simulink model "Horizontal1804"  (R2026b)
settings: Solver=FixedStepDiscrete  StopTime=inf  FixedStep=Official.Step
PostLoadFcn:
  | run(fullfile(fileparts(get_param('StampFly_IMU400','FileName')),'config','startup.m'));
InitFcn:
  | init_imu_flight;
undefined symbols (not defined in the file): Official
libraries: slpidlib x7, simulink x4, mspfiltlib x1
(part 2 of 5)

== system Horizontal1804/JoystickCommand ==
  BasicJoystick : MATLABSystem  Description=公式 Atom JoyStick の指令を ESP-NOW で受信します。Stick6 は [Roll, Pitch, Yaw, Thrust, 制御モード, 高度モード]。アーム、通信状態、姿勢リセット、新パケット、エラーも出力します。Flip 用ボタンは無視します。Channel は自分専用の 1～13 にし、機体のログ送信・受信機と揃えます。  Priority=5  System=basic.Joystick400  SampleTime=.0025  Channel=uint8( 3 )  SimulateUsing=Code generation
      mask Type: basic.Joystick400
  JoystickCommandBus : BusCreator  Description=JoystickCommandBus：異なる単位・型を持つ関連信号を名前付きバスにまとめます。入力線の信号名が項目名です。  Inputs=4  OutDataTypeStr=Bus: BasicLogPilotBus  NonVirtualBus=on
  RadioDiagnosticsBus : BusCreator  Description=RadioDiagnosticsBus：異なる単位・型を持つ関連信号を名前付きバスにまとめます。入力線の信号名が項目名です。  Inputs=2
  RadioDiagnosticsFields : BusSelector  Description=RadioDiagnosticsFields：バスから LinkAge,PacketError を選びます。元のベクトルの成分順序は変更しません。  OutputSignals=LinkAge,PacketError
  RawRadioAgeUnused : Terminator
      settings: Description=RawRadioAgeUnused：使用しない観測出力をここで終端します。接続された制御信号を変更しません。
  JoystickCommand : Outport
  tag scope: JoystickPacketError=global, JoystickPilot=global
  wires:
  RadioDiagnosticsBus/1 -> RadioDiagnosticsFields/1  "RadioDiagnostics"
  BasicJoystick/6 -> RadioDiagnosticsBus/2  "PacketError"
  BasicJoystick/1 -> JoystickCommandBus/1  "Sticks"
  BasicJoystick/5 -> JoystickCommandBus/3  "NewPacket"
  BasicJoystick/2 -> JoystickCommandBus/2  "ArmButton"
  BasicJoystick/3 -> RadioDiagnosticsBus/1  "LinkAge"
  JoystickCommandBus/1 -> JoystickCommand/1, [JoystickPilot]  "JoystickCommand"
  BasicJoystick/4 -> JoystickCommandBus/4  "AHRSRequest"
  RadioDiagnosticsFields/1 -> RawRadioAgeUnused/1  "<LinkAge>"
  RadioDiagnosticsFields/2 -> [JoystickPacketError]  "<PacketError>"

== system Horizontal1804/JoystickFeedback40 ==
  JapaneseExplanation : Subsystem  Description=公式 JoyStick の画面へ姿勢・高度・電池・制御状態を 40 Hz で返信します。通常ログとは別の公式 120 byte 形式です。
      mask help: 公式 JoyStick の画面へ姿勢・高度・電池・制御状態を 40 Hz で返信します。通常ログとは別の公式 120 byte 形式です。
      mask Display: disp(sprintf('公式 JoyStick の画面へ姿勢・高度・電池・制御状態を 40 Hz で返信します。\n通常ログとは別の公式 120 byte 形式です。'));
  OfficialHeaderGains20 : Constant  Description=OfficialHeaderGains20：固定値 single([.65;.7;.01;.125;.95;.7;.025;.125;3;.8;.01;.125;5;4;.04;.125;5;4;.04;.125]) を出力します。意味と単位は親の機能説明と信号名を参照します。  Value=single([.65;.7;.01;.125;.95;.7;.025;.125;3;.8;.01;.125;5;4;.04;.125;5;4;.04;.125])
  OfficialJoyTelemetry40 : MATLABSystem  Description=公式の 27 float 値とゲイン表、高度モード、飛行モード、前方距離を 40 Hz で JoyStick へ返信します。公式 120 byte 形式を保ちます。Sent は送信要求の結果です。  Priority=240  System=official.RadioTelemetryWrite40  SimulateUsing=Code generation
      mask Type: official.RadioTelemetryWrite40
  OfficialTelemetryValues : MATLAB Function  Description=JoyStick へ返す公式 120 byte テレメトリの 27 個の float 値を作ります。時刻・姿勢・目標・電池・加速度・速度・高度などを公式の単位と順序へ変換します。送信は後段の専用 I/O ブロックが行います。  TreatAsAtomicUnit=on
  Sent : Outport
  wires:
  [MotorDuty] -> OfficialTelemetryValues/8(arg_duty)
  [ControlDiagnostics] -> OfficialTelemetryValues/5(arg_cd)
  [FilteredAngularRate] -> OfficialTelemetryValues/4(arg_r)
  [AttitudeAngles] -> OfficialTelemetryValues/3(arg_a)
  [SamplePeriod] -> OfficialTelemetryValues/2(arg_dt)
  [TimeSeconds] -> OfficialTelemetryValues/1(arg_t)
  [BatteryVoltage] -> OfficialTelemetryValues/7(arg_voltage)
  [RawAcceleration] -> OfficialTelemetryValues/6(arg_accel)
  [EstimatedAltitude] -> OfficialTelemetryValues/9(arg_z)
  [SensorDiagnostics] -> OfficialTelemetryValues/10(arg_sd)
  [VerticalVelocity] -> OfficialTelemetryValues/11(arg_v)
  OfficialTelemetryValues/1(arg_values) -> OfficialJoyTelemetry40/1
  OfficialHeaderGains20/1 -> OfficialJoyTelemetry40/2
  [UnusedFrontRangeMm] -> OfficialJoyTelemetry40/5
  [AltitudeEnabled] -> OfficialJoyTelemetry40/3
  [FlightMode] -> OfficialJoyTelemetry40/4
  OfficialJoyTelemetry40/1 -> Sent/1

== system Horizontal1804/LEDAndBuzzer ==
  ControlMode : Selector  Description=ControlMode：必要なベクトル成分を選びます。選択位置は設定画面の Indices で確認します。  InputPortWidth=6  IndexOptions=Index vector (dialog)  Indices=5  OutputSizes=1
  LowVoltageCount : Selector  Description=LowVoltageCount：必要なベクトル成分を選びます。選択位置は設定画面の Indices で確認します。  InputPortWidth=3  IndexOptions=Index vector (dialog)  Indices=3  OutputSizes=1
  StatusIndicators : MATLAB Function  Description=飛行モード・電池・通信状態を LED 色とブザーへ変換します。待ち時間は 400 Hz のカウンターで管理し、機体ボタンの押下・解放を確認して再起動要求を出します。実際の LED・音・再起動は後段の I/O が行います。  TreatAsAtomicUnit=on
  StatusWrite : MATLABSystem  Description=RGB 色 2 個、ブザー周波数 [Hz]、再起動要求を機体の出力キューへ渡します。LED・音の更新は別タスクで実行します。再起動要求は機体の再起動に直結するので、状態判定ブロックからの信号を接続します。  System=official.StatusWrite400  SimulateUsing=Code generation
      mask Type: official.StatusWrite400
  UserButton : MATLABSystem  Description=StampS3 の GPIO0 ボタンを読み、押下中は uint8(1) を出力します。操縦用 JoyStick のボタンとは別です。押下時間と解放の判定は StatusIndicators で行います。  System=official.UserButton400  SimulateUsing=Code generation
      mask Type: official.UserButton400
  wires:
  [AttitudeResetRequest] -> StatusIndicators/6(arg_ahrsFlag)
  LowVoltageCount/1 -> StatusIndicators/4(arg_lowVoltage)
  [SensorFlags] -> LowVoltageCount/1
  [JoystickSticks] -> ControlMode/1
  [JoystickPacketError] -> StatusIndicators/5(arg_rcError)
  [AltitudeEnabled] -> StatusIndicators/3(arg_altFlag)
  [PreviousMode] -> StatusIndicators/1(arg_mode)
  ControlMode/1 -> StatusIndicators/2(arg_controlMode)
  UserButton/1 -> StatusIndicators/7(arg_button)
  StatusIndicators/1(arg_color1) -> StatusWrite/1
  StatusIndicators/2(arg_color2) -> StatusWrite/2
  StatusIndicators/3(arg_tone) -> StatusWrite/3
  StatusIndicators/4(arg_restart) -> StatusWrite/4

== system Horizontal1804/MagnetometerSensor ==
  DeviceRead : MATLABSystem  Description=BMM150 の補償済み磁場 XYZ [μT]、有効性・Fresh・エラー、診断を出力します。新規測定は約 30 Hz、モデルは 400 Hz で最新値を受け取ります。ToF・電池と I2C 排他を共有します。磁気は表示・記録用です。  System=stampfly.BMM150  I2CAddress=uint8( 16 )  SampleTime=.0025  SimulateUsing=Code generation
      mask Type: stampfly.BMM150
  JapaneseExplanation : Subsystem  Description=BMM150 の磁場 XYZ [μT] と有効性・Fresh・診断を取得します。センサー座標を保ってログへ渡し、姿勢推定・制御には使いません。
      mask help: BMM150 の磁場 XYZ [μT] と有効性・Fresh・診断を取得します。センサー座標を保ってログへ渡し、姿勢推定・制御には使いません。
      mask Display: disp(sprintf('BMM150 の磁場 XYZ [μT] と有効性・Fresh・診断を取得します。\nセンサー座標を保ってログへ渡し、姿勢推定・制御には使いません。'));
  SensorDataBus : BusCreator  Description=SensorDataBus：異なる単位・型を持つ関連信号を名前付きバスにまとめます。入力線の信号名が項目名です。  Inputs=3  OutDataTypeStr=Bus: LogMagBus  NonVirtualBus=on
  MagneticField : Outport
  wires:
  SensorDataBus/1 -> MagneticField/1  "SensorData"
  DeviceRead/1 -> SensorDataBus/1  "Field"
  DeviceRead/2 -> SensorDataBus/2  "Flags"
  DeviceRead/3 -> SensorDataBus/3  "Info"

== system Horizontal1804/ModelExplanation ==

== system Horizontal1804/MotorWrite ==
  MotorCommand : Inport
  JapaneseExplanation : Subsystem  Description=8 bit の Counts を実機モーターへ適用します。順序 [FR, FL, RR, RL]、GPIO [42, 5, 41, 10]、150 kHz 指定です。実適用 Counts と PWM 診断を Goto で公開します。
      mask help: 8 bit の Counts を実機モーターへ適用します。順序 [FR, FL, RR, RL]、GPIO [42, 5, 41, 10]、150 kHz 指定です。実適用 Counts と PWM 診断を Goto で公開します。
      mask Display: disp(sprintf('8 bit の Counts を実機モーターへ適用します。\n順序 [FR, FL, RR, RL]、GPIO [42, 5, 41, 10]、150 kHz 指定です。\n実適用 Counts と PWM 診断を Goto で公開します。'));
  MotorCommandFields : BusSelector  Description=MotorCommandFields：バスから Duty,Counts を選びます。元のベクトルの成分順序は変更しません。  OutputSignals=Duty,Counts
  MotorOutputEnabled : Constant  Description=MotorOutputEnabled：固定値 true を出力します。意味と単位は親の機能説明と信号名を参照します。  Value=true  SampleTime=Official.Step
  PWM150kHz8bit : MATLABSystem  Description=入力 Counts4 は [FR, FL, RR, RL] の 8 bit PWM カウントです。Enable と AllowMotorOutput が有効なとき実機へ適用し、実適用値と状態を返します。機体用は 150 kHz 指定です。これは回転数の測定値ではありません。  Priority=100  System=official.MotorPWM400  SampleTime=Official.Step  AllowMotorOutput=true  SimulateUsing=Code generation
      mask Type: official.MotorPWM400
  AppliedCounts : Outport
  PWMStatus : Outport  Port=2
  tag scope: AppliedPWMCounts=global, MotorDuty=global, PWMStatus=global
  wires:
  PWM150kHz8bit/2 -> [PWMStatus], PWMStatus/1
  MotorCommandFields/1 -> [MotorDuty]  "<Duty>"
  MotorCommand/1 -> MotorCommandFields/1
  MotorCommandFields/2 -> PWM150kHz8bit/1  "<Counts>"
  MotorOutputEnabled/1 -> PWM150kHz8bit/2
  PWM150kHz8bit/1 -> AppliedCounts/1, [AppliedPWMCounts]

== system Horizontal1804/OpticalFlowDistance50 ==
  OpticalFlow : Inport
  Attitude : Inport  Port=2
  BottomRange : Inport  Port=3
  RawIMU : Inport  Port=4
  AttitudeFields : BusSelector  Description=AttitudeFields：バスから Angles を選びます。元のベクトルの成分順序は変更しません。  OutputSignals=Angles
  DistanceData : BusCreator  Description=DistanceData：異なる単位・型を持つ関連信号を名前付きバスにまとめます。入力線の信号名が項目名です。  Inputs=3  OutDataTypeStr=Bus: LogDistanceBus  NonVirtualBus=on
  FlowFields : BusSelector  Description=FlowFields：バスから Totals,Raw を選びます。元のベクトルの成分順序は変更しません。  OutputSignals=Totals,Raw
  GroundMotionDistance : MATLABSystem  Description=400 Hz の累積カウント差を 50 Hz で集計し、姿勢・ToF・角速度を使って平らな床上の [東, 北] 移動距離 [m] に換算します。不適切な区間は位置を保持します。385 count/rad は校正前の初期値です。出力は表示・記録専用です。  System=imu.FlowDistance50  SampleTime=0.02  XCountsPerRad=385  YCountsPerRad=385  MinQuality=25  MaxHeightM=2  MaxHorizontalSpeedMps=1.5  MaxVerticalSpeedMps=2  MinDownProjection=0.5  SimulateUsing=Code generation
      mask Type: imu.FlowDistance50
  IMUFields : BusSelector  Description=IMUFields：バスから AngularRate を選びます。元のベクトルの成分順序は変更しません。  OutputSignals=AngularRate
  JapaneseExplanation : Subsystem  Description=生の累積光学フロー、姿勢、角速度、下向き ToF から平面上の東・北移動距離を 50 Hz で作ります。回転補償と品質判定を行い、無効な区間は位置を保持します。385 count/rad は初期値です。
      mask help: 生の累積光学フロー、姿勢、角速度、下向き ToF から平面上の東・北移動距離を 50 Hz で作ります。回転補償と品質判定を行い、無効な区間は位置を保持します。385 count/rad は初期値です。
      mask Display: disp(sprintf('生の累積光学フロー、姿勢、角速度、下向き ToF から平面上の東・北移動距離を 50 Hz で作ります\n。\n回転補償と品質判定を行い、無効な区間は位置を保持します。\n385 count/rad は初期値です。'));
  MillimetersToMeters : Gain  Description=MillimetersToMeters：入力に single(.001) を掛けます。座標変換・単位換算・制御係数は用途ごとに維持します。  Gain=single(.001)
  PoseAndRange4 : Mux  Description=PoseAndRange4：同じ型の値を入力端子の順でベクトルに結合します。ログ仕様・モーター順に対応する結合は順序を保ちます。  Inputs=2
  RangeFields : BusSelector  Description=RangeFields：バスから DistanceMm を選びます。元のベクトルの成分順序は変更しません。  OutputSignals=DistanceMm
  RangeToSingle : DataTypeConversion  Description=RangeToSingle：後段のバス・演算に合わせて single 型へ変換します。  OutDataTypeStr=single  SaturateOnIntegerOverflow=off  RndMeth=Floor
  FlowDistance : Outport
  wires:
  OpticalFlow/1 -> FlowFields/1  "OpticalFlow"
  RangeFields/1 -> RangeToSingle/1  "<DistanceMm>"
  BottomRange/1 -> RangeFields/1  "BottomRange"
  RawIMU/1 -> IMUFields/1  "RawIMU"
  Attitude/1 -> AttitudeFields/1  "Attitude"
  RangeToSingle/1 -> MillimetersToMeters/1
  MillimetersToMeters/1 -> PoseAndRange4/2  "ToFRangeM"
  AttitudeFields/1 -> PoseAndRange4/1  "<Angles>"
  FlowFields/1 -> GroundMotionDistance/1  "<Totals>"
  FlowFields/2 -> GroundMotionDistance/2  "<Raw>"
  IMUFields/1 -> GroundMotionDistance/3  "<AngularRate>"
  PoseAndRange4/1 -> GroundMotionDistance/4  "PoseAndRange"
  GroundMotionDistance/1 -> DistanceData/1  "PositionEN"
  GroundMotionDistance/2 -> DistanceData/2  "Used"
  GroundMotionDistance/3 -> DistanceData/3  "DeltaEN"
  DistanceData/1 -> FlowDistance/1  "FlowDistance"

== system Horizontal1804/OpticalFlowSensor ==
  DeviceRead : MATLABSystem  Description=SPI の Motion Burst から 2 軸の差分カウント、品質 Raw8、診断 Info4、巡回する累積 Totals2 を 400 Hz で取得します。カウントは距離・速度そのものではありません。距離換算は後段の FlowDistance50 で行います。  System=stampfly.PMW3901MB  SampleTime=.0025  SimulateUsing=Code generation
      mask Type: stampfly.PMW3901MB
  JapaneseExplanation : Subsystem  Description=PMW3901 の生 2 軸差分・品質・診断・累積カウントを取得します。表示・記録専用で、水平位置制御へは戻しません。
      mask help: PMW3901 の生 2 軸差分・品質・診断・累積カウントを取得します。表示・記録専用で、水平位置制御へは戻しません。
      mask Display: disp(sprintf('PMW3901 の生 2 軸差分・品質・診断・累積カウントを取得します。\n表示・記録専用で、水平位置制御へは戻しません。'));
  SensorDataBus : BusCreator  Description=SensorDataBus：異なる単位・型を持つ関連信号を名前付きバスにまとめます。入力線の信号名が項目名です。  Inputs=4  OutDataTypeStr=Bus: LogFlowBus  NonVirtualBus=on
  OpticalFlow : Outport
  wires:
  DeviceRead/1 -> SensorDataBus/1  "Delta"
  DeviceRead/2 -> SensorDataBus/2  "Raw"
  DeviceRead/3 -> SensorDataBus/3  "Info"
  DeviceRead/4 -> SensorDataBus/4  "Totals"
  SensorDataBus/1 -> OpticalFlow/1  "SensorData"

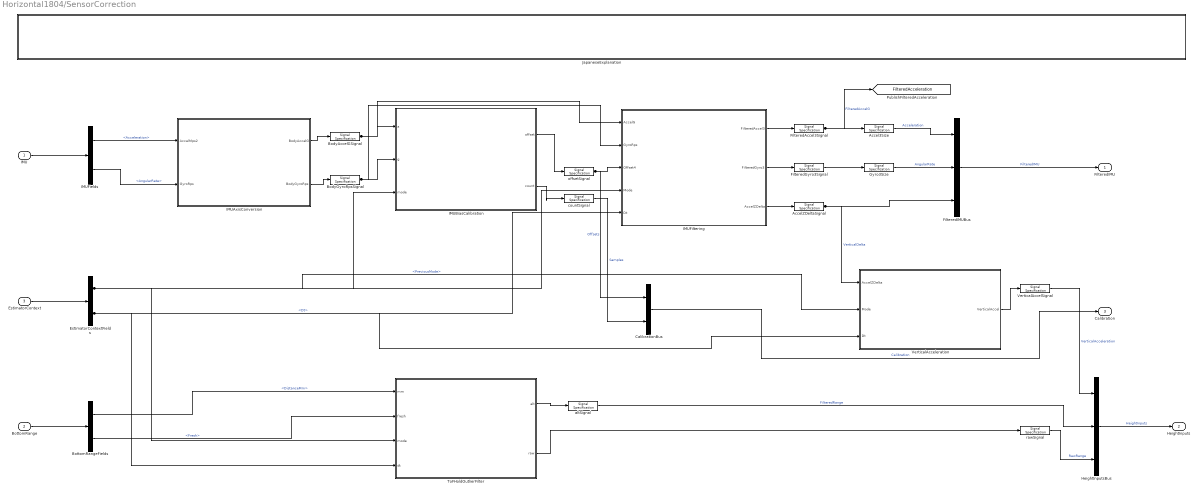
== system Horizontal1804/SensorCorrection ==
  IMU : Inport
  BottomRange : Inport  Port=2
  EstimatorContext : Inport  Port=3
  Accel3Size : SignalSpecification  OutDataTypeStr=single  Dimensions=3
  AccelZDeltaSignal : SignalSpecification  OutDataTypeStr=single  Dimensions=1
  BodyAccelGSignal : SignalSpecification  OutDataTypeStr=single  Dimensions=3
  BodyGyroRpsSignal : SignalSpecification  OutDataTypeStr=single  Dimensions=3
  BottomRangeFields : BusSelector  Description=BottomRangeFields：バスから DistanceMm,Fresh を選びます。元のベクトルの成分順序は変更しません。  OutputSignals=DistanceMm,Fresh
  CalibrationBus : BusCreator  Description=CalibrationBus：異なる単位・型を持つ関連信号を名前付きバスにまとめます。入力線の信号名が項目名です。  Inputs=2
  EstimatorContextFields : BusSelector  Description=EstimatorContextFields：バスから PreviousMode,Dt を選びます。元のベクトルの成分順序は変更しません。  OutputSignals=PreviousMode,Dt
  FilteredAccel3Signal : SignalSpecification  OutDataTypeStr=single  Dimensions=3
  FilteredGyro3Signal : SignalSpecification  OutDataTypeStr=single  Dimensions=3
  FilteredIMUBus : BusCreator  Description=FilteredIMUBus：異なる単位・型を持つ関連信号を名前付きバスにまとめます。入力線の信号名が項目名です。  Inputs=3
  Gyro3Size : SignalSpecification  OutDataTypeStr=single  Dimensions=3
  HeightInputsBus : BusCreator  Description=HeightInputsBus：異なる単位・型を持つ関連信号を名前付きバスにまとめます。入力線の信号名が項目名です。  Inputs=3
  IMUAxisConversion : Subsystem  Description=センサー XYZ を機体 [Y, X, -Z] へ変換します。加速度を m/s² から g 基準へ換算し、角速度は rad/s を保ちます。この座標変換はセンサーの取り付けと既存制御の定義に必要です。
      mask help: センサー XYZ を機体 [Y, X, -Z] へ変換します。加速度を m/s² から g 基準へ換算し、角速度は rad/s を保ちます。この座標変換はセンサーの取り付けと既存制御の定義に必要です。
      mask Display: disp('IMUAxisConversion');port_label('input',1,'AccelMps2');port_label('input',2,'GyroRps');port_label('output',1,'BodyAccelG');port_label('output',2,'BodyGyroRps');
  IMUBiasCalibration : MATLAB Function  Description=起動時に静止した機体のジャイロ XYZ と加速度 Z を 800 周期平均します。出力 Offset は [GyroX; GyroY; GyroZ; AccelZ]、Count は取得数です。400 Hz で公称 2 秒の校正中は機体を動かさないでください。  TreatAsAtomicUnit=on
  IMUFields : BusSelector  Description=IMUFields：バスから Acceleration,AngularRate を選びます。元のベクトルの成分順序は変更しません。  OutputSignals=Acceleration,AngularRate
  IMUFiltering : Subsystem  Description=加速度と校正後角速度の XYZ ベクトルを時定数 3 ms で低域フィルターに通します。Z 加速度の校正差分は 100 ms で処理します。Mode 0, 1 の保持、待機への移行時リセット、実測 dt と既存の演算順序を維持します。
      mask help: 加速度と校正後角速度の XYZ ベクトルを時定数 3 ms で低域フィルターに通します。Z 加速度の校正差分は 100 ms で処理します。Mode 0, 1 の保持、待機への移行時リセット、実測 dt と既存の演算順序を維持します。
      mask Display: disp('IMUFiltering');port_label('input',1,'AccelG');port_label('input',2,'GyroRps');port_label('input',3,'Offset4');port_label('input',4,'Mode');port_label('input',5,'Dt');port_label('output',1,'FilteredAccel3');port_label('output',2,'FilteredGyro3');port_label('output',3,'AccelZDelta');
  JapaneseExplanation : Subsystem  Description=センサー座標から機体 XYZ へ変換し、800 周期の静止校正とフィルターを行います。加速度 XYZ・角速度 XYZ の順を維持し、ToF の保持・外れ値処理と鉛直加速度もまとめます。推定用の前処理は Mode 0, 1 で保持します。
      mask help: センサー座標から機体 XYZ へ変換し、800 周期の静止校正とフィルターを行います。加速度 XYZ・角速度 XYZ の順を維持し、ToF の保持・外れ値処理と鉛直加速度もまとめます。推定用の前処理は Mode 0, 1 で保持します。
      mask Display: disp(sprintf('センサー座標から機体 XYZ へ変換し、800 周期の静止校正とフィルターを行います。\n加速度 XYZ・角速度 XYZ の順を維持し、ToF の保持・外れ値処理と鉛直加速度もまとめます。\n推定用の前処理は Mode 0, 1 で保持します。'));
  ToFHoldOutlierFilter : MATLAB Function  Description=新しい下向き距離 [mm] を保持・外れ値処理して高さ [m] へ変換します。20 mm 以下は前回の有効距離を使い、500 mm 超の飛びは最大 2 回まで履歴から補外します。Mode 0, 1 では推定用の出力を保持します。  TreatAsAtomicUnit=on
  VerticalAccelSignal : SignalSpecification  OutDataTypeStr=single  Dimensions=1
  VerticalAcceleration : Subsystem  Description=校正後の Z 加速度差分の符号を反転し、上向きの鉛直加速度を作ります。100 ms の平滑化とモードによる保持・リセットを行います。高度 Kalman は従来の g 基準の数値を受けます。
      mask help: 校正後の Z 加速度差分の符号を反転し、上向きの鉛直加速度を作ります。100 ms の平滑化とモードによる保持・リセットを行います。高度 Kalman は従来の g 基準の数値を受けます。
      mask Display: disp('VerticalAcceleration');port_label('input',1,'AccelZDelta');port_label('input',2,'Mode');port_label('input',3,'Dt');port_label('output',1,'VerticalAccel');
  altSignal : SignalSpecification  OutDataTypeStr=single  Dimensions=1
  countSignal : SignalSpecification  OutDataTypeStr=uint16  Dimensions=1
  offsetSignal : SignalSpecification  OutDataTypeStr=single  Dimensions=4
  rawSignal : SignalSpecification  OutDataTypeStr=int16  Dimensions=1
  FilteredIMU : Outport
  HeightInputs : Outport  Port=2
  Calibration : Outport  Port=3
  tag scope: FilteredAcceleration=global
  wires:
  EstimatorContext/1 -> EstimatorContextFields/1
  BottomRangeFields/2 -> ToFHoldOutlierFilter/2(fresh)  "<Fresh>"
  IMUAxisConversion/2(BodyGyroRps) -> BodyGyroRpsSignal/1
  IMU/1 -> IMUFields/1
  IMUBiasCalibration/2(count) -> countSignal/1
  IMUFields/1 -> IMUAxisConversion/1(AccelMps2)  "<Acceleration>"
  IMUFields/2 -> IMUAxisConversion/2(GyroRps)  "<AngularRate>"
  BottomRangeFields/1 -> ToFHoldOutlierFilter/1(mm)  "<DistanceMm>"
  IMUAxisConversion/1(BodyAccelG) -> BodyAccelGSignal/1
  FilteredGyro3Signal/1 -> Gyro3Size/1
  BottomRange/1 -> BottomRangeFields/1
  BodyAccelGSignal/1 -> IMUFiltering/1(AccelG), IMUBiasCalibration/1(a)
  HeightInputsBus/1 -> HeightInputs/1  "HeightInputs"
  BodyGyroRpsSignal/1 -> IMUFiltering/2(GyroRps), IMUBiasCalibration/2(g)
  EstimatorContextFields/1 -> IMUFiltering/4(Mode), VerticalAcceleration/2(Mode), ToFHoldOutlierFilter/3(mode), IMUBiasCalibration/3(mode)  "<PreviousMode>"
  EstimatorContextFields/2 -> VerticalAcceleration/3(Dt), IMUFiltering/5(Dt), ToFHoldOutlierFilter/4(dt)  "<Dt>"
  IMUBiasCalibration/1(offset) -> offsetSignal/1
  ToFHoldOutlierFilter/1(alt) -> altSignal/1
  Gyro3Size/1 -> FilteredIMUBus/2  "AngularRate"
  AccelZDeltaSignal/1 -> VerticalAcceleration/1(AccelZDelta), FilteredIMUBus/3  "VerticalDelta"
  ToFHoldOutlierFilter/2(raw) -> rawSignal/1
  countSignal/1 -> CalibrationBus/2  "Samples"
  offsetSignal/1 -> IMUFiltering/3(Offset4), CalibrationBus/1  "Offsets"
  CalibrationBus/1 -> Calibration/1  "Calibration"
  altSignal/1 -> HeightInputsBus/2  "FilteredRange"
  IMUFiltering/1(FilteredAccel3) -> FilteredAccel3Signal/1
  IMUFiltering/2(FilteredGyro3) -> FilteredGyro3Signal/1
  IMUFiltering/3(AccelZDelta) -> AccelZDeltaSignal/1
  VerticalAccelSignal/1 -> HeightInputsBus/1  "VerticalAcceleration"
  rawSignal/1 -> HeightInputsBus/3  "RawRange"
  FilteredAccel3Signal/1 -> [FilteredAcceleration], Accel3Size/1  "FilteredAccelG"
  VerticalAcceleration/1(VerticalAccel) -> VerticalAccelSignal/1
  Accel3Size/1 -> FilteredIMUBus/1  "Acceleration"
  FilteredIMUBus/1 -> FilteredIMU/1  "FilteredIMU"

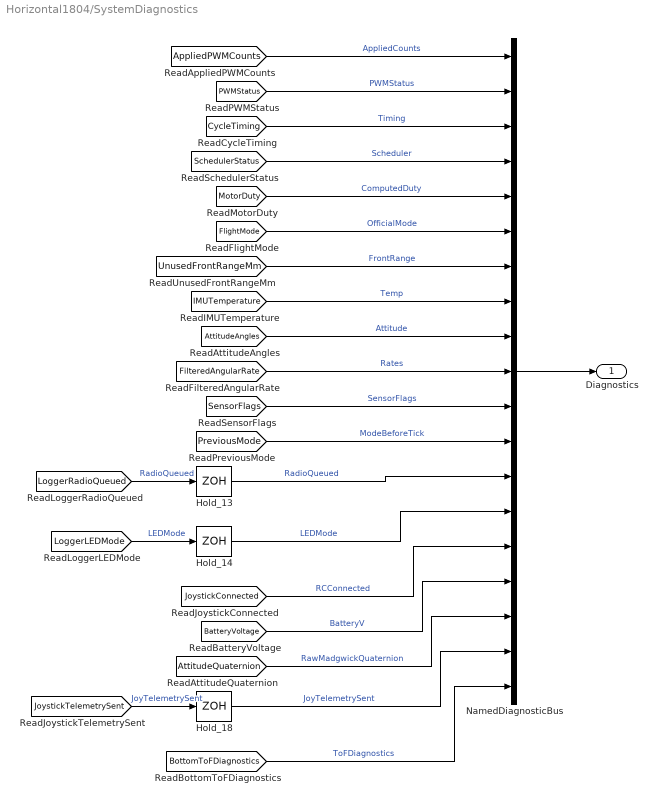
== system Horizontal1804/SystemDiagnostics ==
  Hold_13 : ZeroOrderHold  Description=Hold_13：入力の最新値を指定周期で保持します。異なる更新周期の観測値を診断へ渡します。  SampleTime=.0025
  Hold_14 : ZeroOrderHold  Description=Hold_14：入力の最新値を指定周期で保持します。異なる更新周期の観測値を診断へ渡します。  SampleTime=.0025
  Hold_18 : ZeroOrderHold  Description=Hold_18：入力の最新値を指定周期で保持します。異なる更新周期の観測値を診断へ渡します。  SampleTime=.0025
  NamedDiagnosticBus : BusCreator  Description=NamedDiagnosticBus：異なる単位・型を持つ関連信号を名前付きバスにまとめます。入力線の信号名が項目名です。  Inputs=19  OutDataTypeStr=Bus: OfficialDiagnosticBus  NonVirtualBus=on
  Diagnostics : Outport
  wires:
  [SchedulerStatus] -> NamedDiagnosticBus/4  "Scheduler"
  [AppliedPWMCounts] -> NamedDiagnosticBus/1  "AppliedCounts"
  [LoggerRadioQueued] -> Hold_13/1  "RadioQueued"
  [LoggerLEDMode] -> Hold_14/1  "LEDMode"
  [PWMStatus] -> NamedDiagnosticBus/2  "PWMStatus"
  [JoystickTelemetrySent] -> Hold_18/1  "JoyTelemetrySent"
  [MotorDuty] -> NamedDiagnosticBus/5  "ComputedDuty"
  [CycleTiming] -> NamedDiagnosticBus/3  "Timing"
  [FlightMode] -> NamedDiagnosticBus/6  "OfficialMode"
  [UnusedFrontRangeMm] -> NamedDiagnosticBus/7  "FrontRange"
  [IMUTemperature] -> NamedDiagnosticBus/8  "Temp"
  [AttitudeAngles] -> NamedDiagnosticBus/9  "Attitude"
  [FilteredAngularRate] -> NamedDiagnosticBus/10  "Rates"
  [SensorFlags] -> NamedDiagnosticBus/11  "SensorFlags"
  [PreviousMode] -> NamedDiagnosticBus/12  "ModeBeforeTick"
  Hold_13/1 -> NamedDiagnosticBus/13  "RadioQueued"
  Hold_14/1 -> NamedDiagnosticBus/14  "LEDMode"
  [JoystickConnected] -> NamedDiagnosticBus/15  "RCConnected"
  [BatteryVoltage] -> NamedDiagnosticBus/16  "BatteryV"
  [AttitudeQuaternion] -> NamedDiagnosticBus/17  "RawMadgwickQuaternion"
  Hold_18/1 -> NamedDiagnosticBus/18  "JoyTelemetrySent"
  [BottomToFDiagnostics] -> NamedDiagnosticBus/19  "ToFDiagnostics"
  NamedDiagnosticBus/1 -> Diagnostics/1

== system Horizontal1804/TickStart ==
  CycleClock : MATLABSystem  Description=2500 μs の GPTimer で制御タスクを起動し、開始時刻 [μs]、実測 dt [s]、タイマー診断を返します。モデルの Fixed-step も 0.0025 秒に揃えます。生成された step の計測設定はモデル名 StampFly_IMU400 に対応しています。  Priority=1  System=official.TickStart400  SampleTime=Official.Step  SimulateUsing=Code generation
      mask Type: official.TickStart400
  UsToSeconds : Gain  Description=UsToSeconds：入力に single(1e-6) を掛けます。座標変換・単位換算・制御係数は用途ごとに維持します。  Gain=single(1e-6)  OutDataTypeStr=single
  Dt : Outport
  tag scope: CycleStartUs=global, SamplePeriod=global, SchedulerStatus=global, TimeSeconds=global
  wires:
  CycleClock/1 -> [CycleStartUs], UsToSeconds/1  "StartUs"
  CycleClock/2 -> Dt/1, [SamplePeriod]
  CycleClock/3 -> [SchedulerStatus]
  UsToSeconds/1 -> [TimeSeconds]

== system Horizontal1804/AttitudeAltitudeEstimation/IMUAttitude ==
  AngularRate : Inport
  AccelerationG : Inport  Port=2
  PreviousMode : Inport  Port=3
  AttitudeReset : Inport  Port=4
  FilterInputs : MATLAB Function  Description=IMU Filter の入力を準備します。機体座標 XYZ の角速度 [rad/s] と加速度 [g] を、推定器の座標と SI 単位へ変換します。校正中のリセット要求は、推定を再開するまで保持します。  TreatAsAtomicUnit=on
  FlightOutputs : MATLAB Function  Description=IMU Filter の姿勢とバイアス補正済み角速度を、従来の飛行制御の座標・順序へ戻します。出力は角度 [Roll, Pitch, Yaw] [rad]、クォータニオン [w, x, y, z]、機体 XYZ 角速度 [rad/s] です。  TreatAsAtomicUnit=on
  FusionState : Subsystem  Description=Mode 0, 1 では IMU Filter の予測・補正を実行せず状態を保持する Enabled subsystem です。停止中のリセットは FilterInputs が記憶し、再開時に内部へ渡します。  TreatAsAtomicUnit=on
      mask help: Mode 0, 1 では IMU Filter の予測・補正を実行せず状態を保持する Enabled subsystem です。停止中のリセットは FilterInputs が記憶し、再開時に内部へ渡します。
      mask Display: disp('FusionState');port_label('input',1,'Accel');port_label('input',2,'Gyro');port_label('input',3,'Reset');port_label('output',1,'Orientation');port_label('output',2,'AngularVelocity');
  Angles : Outport
  Quaternion : Outport  Port=2
  CorrectedAngularRate : Outport  Port=3
  wires:
  AngularRate/1 -> FlightOutputs/5(rawRates), FilterInputs/1(rates)
  AccelerationG/1 -> FilterInputs/2(accelG)
  FilterInputs/4(filterReset) -> FusionState/3(Reset)  "PendingReset"
  AttitudeReset/1 -> FilterInputs/4(reset), FlightOutputs/4(reset)
  FilterInputs/3(run) -> FusionState/Enable, FlightOutputs/3(run)
  FilterInputs/2(gyroRps) -> FusionState/2(Gyro)  "GyroRps"
  PreviousMode/1 -> FilterInputs/3(mode)
  FilterInputs/1(accelMps2) -> FusionState/1(Accel)  "AccelMps2"
  FusionState/1(Orientation) -> FlightOutputs/1(orientation)
  FusionState/2(AngularVelocity) -> FlightOutputs/2(angularVelocity)
  FlightOutputs/1(angles) -> Angles/1  "Angles"
  FlightOutputs/2(q) -> Quaternion/1  "Quaternion"
  FlightOutputs/3(rates) -> CorrectedAngularRate/1  "AngularRate"

== system Horizontal1804/AttitudeAltitudeEstimation/JapaneseExplanation ==

== system Horizontal1804/BottomRangeSensor/JapaneseExplanation ==

== system Horizontal1804/CommandPreparation/JapaneseExplanation ==

== system Horizontal1804/DataLogging50/JapaneseExplanation ==

== system Horizontal1804/EstimatorContext/JapaneseExplanation ==

== system Horizontal1804/FlightControl/JapaneseExplanation ==

== system Horizontal1804/FlightControl/PreviousCycle ==
  ControlState : Inport
  SupervisorReset : Inport  Port=2
  AHRSResetMemory : UnitDelay  Description=AHRSResetMemory：前周期の値を保持して出力します。更新順序と状態保持に必要な 1 周期遅延です。初期値 false、周期 Official.Step 秒。  InitialCondition=false  SampleTime=Official.Step
  AltFlagMemory : UnitDelay  Description=AltFlagMemory：前周期の値を保持して出力します。更新順序と状態保持に必要な 1 周期遅延です。初期値 uint8(0)、周期 Official.Step 秒。  InitialCondition=uint8(0)  SampleTime=Official.Step
  AltFlagUInt8 : DataTypeConversion  Description=AltFlagUInt8：後段のバス・演算に合わせて uint8 型へ変換します。  OutDataTypeStr=uint8  SaturateOnIntegerOverflow=off  RndMeth=Floor
  ControlStateFields : BusSelector  Description=ControlStateFields：バスから AltitudeEnabled,Mode を選びます。元のベクトルの成分順序は変更しません。  OutputSignals=AltitudeEnabled,Mode
  EstimatorFeedbackBus : BusCreator  Description=EstimatorFeedbackBus：異なる単位・型を持つ関連信号を名前付きバスにまとめます。入力線の信号名が項目名です。  Inputs=4
  ModeMemory : UnitDelay  Description=ModeMemory：前周期の値を保持して出力します。更新順序と状態保持に必要な 1 周期遅延です。初期値 uint8(0)、周期 Official.Step 秒。  InitialCondition=uint8(0)  SampleTime=Official.Step
  ParkingResetMemory : UnitDelay  Description=ParkingResetMemory：前周期の値を保持して出力します。更新順序と状態保持に必要な 1 周期遅延です。初期値 false、周期 Official.Step 秒。  InitialCondition=false  SampleTime=Official.Step
  SupervisorResetFields : BusSelector  Description=SupervisorResetFields：バスから AttitudeReset,ParkingReset を選びます。元のベクトルの成分順序は変更しません。  OutputSignals=AttitudeReset,ParkingReset
  EstimatorFeedback : Outport
  PreviousMode : Outport  Port=2
  AltitudeEnabled : Outport  Port=3
  wires:
  ControlStateFields/1 -> AltFlagUInt8/1  "<AltitudeEnabled>"
  SupervisorResetFields/1 -> AHRSResetMemory/1  "<AttitudeReset>"
  AltFlagMemory/1 -> EstimatorFeedbackBus/2  "AltitudeEnabled"
  ModeMemory/1 -> EstimatorFeedbackBus/1, PreviousMode/1  "PreviousMode"
  SupervisorReset/1 -> SupervisorResetFields/1
  ControlState/1 -> ControlStateFields/1
  ControlStateFields/2 -> ModeMemory/1  "<Mode>"
  SupervisorResetFields/2 -> ParkingResetMemory/1  "<ParkingReset>"
  ParkingResetMemory/1 -> EstimatorFeedbackBus/4  "ParkingReset"
  AltFlagUInt8/1 -> AltFlagMemory/1, AltitudeEnabled/1  "AltitudeEnabled"
  EstimatorFeedbackBus/1 -> EstimatorFeedback/1  "EstimatorFeedback"
  AHRSResetMemory/1 -> EstimatorFeedbackBus/3  "AttitudeReset"

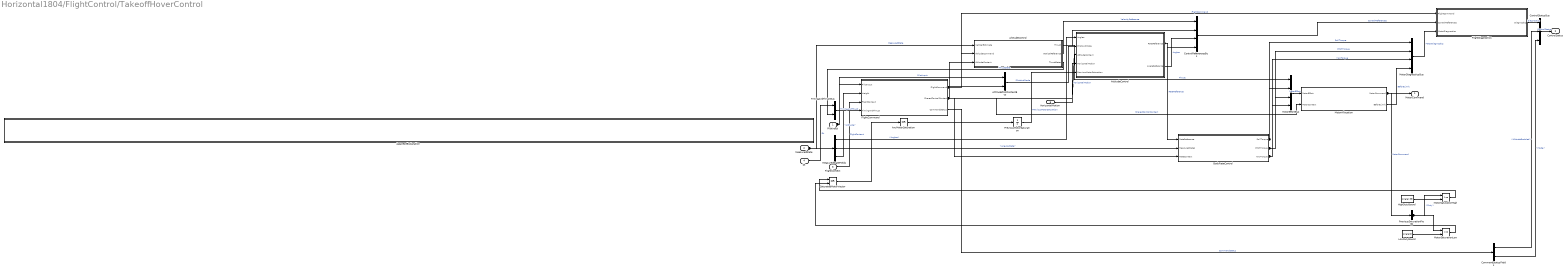
== system Horizontal1804/FlightControl/TakeoffHoverControl ==
  PilotInput : Inport
  MeasuredState : Inport  Port=2
  FlightContext : Inport  Port=3
  Dt : Inport  Port=4
  HorizontalMotion : Inport  Description=HorizontalMotion：水平推定・制御のデータと実行条件を選択・結合します。2軸の順序は局所X（基準機首）、Y（右）です。  Port=5  OutDataTypeStr=Bus: HorizontalMotionBus
  AltitudeControl : Subsystem  Description=高度誤差を高度 PID で目標鉛直速度へ変換し、鉛直速度 PID で共通推力を補正します。自動高度と着陸降下を選び、平滑化と推力制限を行います。
      mask help: 高度誤差を高度 PID で目標鉛直速度へ変換し、鉛直速度 PID で共通推力を補正します。自動高度と着陸降下を選び、平滑化と推力制限を行います。
      mask Display: disp('AltitudeControl');port_label('input',1,'VerticalEstimate');port_label('input',2,'AltitudeCommand');port_label('input',3,'AltitudeContext');port_label('output',1,'Thrust');port_label('output',2,'VerticalReference');port_label('output',3,'ThrustState');
  AnyMotorSaturation : Logic  Description=AnyMotorSaturation：水平推定・制御のデータと実行条件を選択・結合します。2軸の順序は局所X（基準機首）、Y（右）です。  Operator=OR  Inputs=1  IconShape=distinctive  AllPortsSameDT=off  OutDataTypeStr=boolean
  AttitudeControl : Subsystem  Description=Stabilize の Roll/Pitch 角度誤差を角度 PID へ渡して角速度目標を作ります。Sport は直接角速度目標を使い、Yaw の指令は角度ループを通しません。
      mask help: Stabilize の Roll/Pitch 角度誤差を角度 PID へ渡して角速度目標を作ります。Sport は直接角速度目標を使い、Yaw の指令は角度ループを通しません。
      mask Display: disp('AttitudeControl');port_label('input',1,'Angles');port_label('input',2,'PilotAndMode');port_label('input',3,'AttitudeContext');port_label('input',4,'HorizontalMotion');port_label('input',5,'PreviousMotorSaturation');port_label('output',1,'RateReference');port_label('output',2,'AngleReference');
  AttitudePilotContextBus : BusCreator  Description=AttitudePilotContextBus：異なる単位・型を持つ関連信号を名前付きバスにまとめます。入力線の信号名が項目名です。  Inputs=2
  BodyRateControl : Subsystem  Description=Roll/Pitch/Yaw の目標と推定角速度との差を各 PID で処理し、モーターに加える 3 軸の補正を作ります。角速度は機体 XYZ、rad/s です。
      mask help: Roll/Pitch/Yaw の目標と推定角速度との差を各 PID で処理し、モーターに加える 3 軸の補正を作ります。角速度は機体 XYZ、rad/s です。
      mask Display: disp('BodyRateControl');port_label('input',1,'RateReference');port_label('input',2,'MeasuredRates');port_label('input',3,'RateContext');port_label('output',1,'RollTorque');port_label('output',2,'PitchTorque');port_label('output',3,'YawTorque');
  CommandStatusFields : BusSelector  Description=CommandStatusFields：バスから AltitudeEnabled,Mode を選びます。元のベクトルの成分順序は変更しません。  OutputSignals=AltitudeEnabled,Mode
  ControlReferencesBus : BusCreator  Description=ControlReferencesBus：異なる単位・型を持つ関連信号を名前付きバスにまとめます。入力線の信号名が項目名です。  Inputs=4
  ControlStatusBus : BusCreator  Description=ControlStatusBus：異なる単位・型を持つ関連信号を名前付きバスにまとめます。入力線の信号名が項目名です。  Inputs=3
  FlightCommand : Subsystem  Description=スティック、高度目標、離着陸カウンター、共通推力とモードを決めます。低推力条件に応じた制御ループの許可・リセットも生成します。
      mask help: スティック、高度目標、離着陸カウンター、共通推力とモードを決めます。低推力条件に応じた制御ループの許可・リセットも生成します。
      mask Display: disp('FlightCommand');port_label('input',1,'PilotInput');port_label('input',2,'Height');port_label('input',3,'FlightContext');port_label('input',4,'TimingAndThrust');port_label('output',1,'FlightCommand');port_label('output',2,'SharedControlContext');port_label('output',3,'CommandStatus');
  FlightDiagnostics : Subsystem  Description=高度目標、推力、角度・角速度目標、3 軸補正、配分前値をログの既存 17 要素順序へまとめます。制御の判断は行いません。
      mask help: 高度目標、推力、角度・角速度目標、3 軸補正、配分前値をログの既存 17 要素順序へまとめます。制御の判断は行いません。
      mask Display: disp('FlightDiagnostics');port_label('input',1,'FlightCommand');port_label('input',2,'ControlReferences');port_label('input',3,'MotorDiagnostics');port_label('output',1,'Diagnostics');
  HighDutyBound : Constant  Description=HighDutyBound：水平推定・制御のデータと実行条件を選択・結合します。2軸の順序は局所X（基準機首）、Y（右）です。  Value=single(.95)
  JapaneseExplanation : Subsystem  Description=離着陸・高度制御・姿勢制御・角速度制御・モーター配分を機能別にまとめます。高度→速度、角度→角速度の二重ループを読みます。
      mask help: 離着陸・高度制御・姿勢制御・角速度制御・モーター配分を機能別にまとめます。高度→速度、角度→角速度の二重ループを読みます。
      mask Display: disp(sprintf('離着陸・高度制御・姿勢制御・角速度制御・モーター配分を機能別にまとめます。\n高度→速度、角度→角速度の二重ループを読みます。'));
  LowDutyBound : Constant  Description=LowDutyBound：水平推定・制御のデータと実行条件を選択・結合します。2軸の順序は局所X（基準機首）、Y（右）です。  Value=single(0)
  MeasuredStateFields : BusSelector  Description=MeasuredStateFields：バスから Angles,AngularRate,Altitude を選びます。元のベクトルの成分順序は変更しません。  OutputSignals=Angles,AngularRate,Altitude
  MotorAllocation : Subsystem  Description=共通推力と 3 軸の補正を [FR, FL, RR, RL] の 4 モーターへ配分します。3 ms 平滑化、Duty 0～0.95 の制限、floor(255*Duty) の量子化を行います。
      mask help: 共通推力と 3 軸の補正を [FR, FL, RR, RL] の 4 モーターへ配分します。3 ms 平滑化、Duty 0～0.95 の制限、floor(255*Duty) の量子化を行います。
      mask Display: disp('MotorAllocation');port_label('input',1,'MotorEffort');port_label('input',2,'MotorContext');port_label('output',1,'MotorCommand');port_label('output',2,'BeforeLimit');
  MotorDiagnosticsBus : BusCreator  Description=MotorDiagnosticsBus：異なる単位・型を持つ関連信号を名前付きバスにまとめます。入力線の信号名が項目名です。  Inputs=4
  MotorEffortBus : BusCreator  Description=MotorEffortBus：異なる単位・型を持つ関連信号を名前付きバスにまとめます。入力線の信号名が項目名です。  Inputs=4
  MotorSaturationHigh : RelationalOperator  Description=MotorSaturationHigh：水平推定・制御のデータと実行条件を選択・結合します。2軸の順序は局所X（基準機首）、Y（右）です。  OutDataTypeStr=boolean  RndMeth=Simplest  InputSameDT=off
  MotorSaturationLow : RelationalOperator  Description=MotorSaturationLow：水平推定・制御のデータと実行条件を選択・結合します。2軸の順序は局所X（基準機首）、Y（右）です。  Operator=<=  OutDataTypeStr=boolean  RndMeth=Simplest  InputSameDT=off
  PreviousMotorSaturation : UnitDelay  Description=PreviousMotorSaturation：水平推定・制御のデータと実行条件を選択・結合します。2軸の順序は局所X（基準機首）、Y（右）です。  InitialCondition=false  SampleTime=Official.Step
  PreviousSaturationFields : BusSelector  Description=PreviousSaturationFields：水平推定・制御のデータと実行条件を選択・結合します。2軸の順序は局所X（基準機首）、Y（右）です。  OutputSignals=Duty
  SaturatedMotorVector : Logic  Description=SaturatedMotorVector：水平推定・制御のデータと実行条件を選択・結合します。2軸の順序は局所X（基準機首）、Y（右）です。  Operator=OR  IconShape=distinctive  AllPortsSameDT=off  OutDataTypeStr=boolean
  TimingAndThrustBus : BusCreator  Description=TimingAndThrustBus：異なる単位・型を持つ関連信号を名前付きバスにまとめます。入力線の信号名が項目名です。  Inputs=2
  MotorCommand : Outport
  ControlStatus : Outport  Port=2
  wires:
  PilotInput/1 -> AttitudePilotContextBus/1, FlightCommand/1(PilotInput)  "PilotInput"
  MeasuredState/1 -> AltitudeControl/1(VerticalEstimate), MeasuredStateFields/1  "MeasuredState"
  AnyMotorSaturation/1 -> PreviousMotorSaturation/1
  SaturatedMotorVector/1 -> AnyMotorSaturation/1
  FlightContext/1 -> FlightCommand/3(FlightContext)  "FlightContext"
  HighDutyBound/1 -> MotorSaturationHigh/2
  MotorDiagnosticsBus/1 -> FlightDiagnostics/3(MotorDiagnostics)  "MotorDiagnostics"
  HorizontalMotion/1 -> AttitudeControl/4(HorizontalMotion)  "HorizontalMotion"
  MeasuredStateFields/3 -> FlightCommand/2(Height)  "<Altitude>"
  Dt/1 -> TimingAndThrustBus/1  "Dt"
  TimingAndThrustBus/1 -> FlightCommand/4(TimingAndThrust)  "TimingAndThrust"
  MeasuredStateFields/1 -> AttitudeControl/1(Angles)  "<Angles>"
  MeasuredStateFields/2 -> BodyRateControl/2(MeasuredRates)  "<AngularRate>"
  FlightCommand/1(FlightCommand) -> FlightDiagnostics/1(FlightCommand), AltitudeControl/2(AltitudeCommand)  "FlightCommand"
  AttitudeControl/1(RateReference) -> BodyRateControl/1(RateReference), ControlReferencesBus/4  "RateReference"
  AltitudeControl/2(VerticalReference) -> ControlReferencesBus/1  "VelocityReference"
  FlightCommand/2(SharedControlContext) -> BodyRateControl/3(RateContext), MotorAllocation/2(MotorContext), AttitudePilotContextBus/2, AltitudeControl/3(AltitudeContext), AttitudeControl/3(AttitudeContext)  "SharedControlContext"
  FlightCommand/3(CommandStatus) -> CommandStatusFields/1  "CommandStatus"
  MotorSaturationHigh/1 -> SaturatedMotorVector/1
  AttitudeControl/2(AngleReference) -> ControlReferencesBus/3  "Angles"
  AltitudeControl/1(Thrust) -> MotorEffortBus/1, ControlReferencesBus/2  "Thrust"
  MotorSaturationLow/1 -> SaturatedMotorVector/2
  AltitudeControl/3(ThrustState) -> TimingAndThrustBus/2  "ThrustState"
  CommandStatusFields/1 -> ControlStatusBus/2  "<AltitudeEnabled>"
  AttitudePilotContextBus/1 -> AttitudeControl/2(PilotAndMode)  "PilotAndMode"
  LowDutyBound/1 -> MotorSaturationLow/2
  BodyRateControl/3(YawTorque) -> MotorDiagnosticsBus/3, MotorEffortBus/4  "YawTorque"
  PreviousMotorSaturation/1 -> AttitudeControl/5(PreviousMotorSaturation)  "PreviousMotorSaturation"
  ControlReferencesBus/1 -> FlightDiagnostics/2(ControlReferences)  "ControlReferences"
  BodyRateControl/1(RollTorque) -> MotorDiagnosticsBus/1, MotorEffortBus/2  "RollTorque"
  BodyRateControl/2(PitchTorque) -> MotorDiagnosticsBus/2, MotorEffortBus/3  "PitchTorque"
  MotorEffortBus/1 -> MotorAllocation/1(MotorEffort)  "MotorEffort"
  MotorAllocation/1(MotorCommand) -> MotorCommand/1, PreviousSaturationFields/1  "MotorCommand"
  MotorAllocation/2(BeforeLimit) -> MotorDiagnosticsBus/4  "BeforeLimit"
  PreviousSaturationFields/1 -> MotorSaturationHigh/1, MotorSaturationLow/1  "<Duty>"
  FlightDiagnostics/1(Diagnostics) -> ControlStatusBus/1  "Diagnostics"
  CommandStatusFields/2 -> ControlStatusBus/3  "<Mode>"
  ControlStatusBus/1 -> ControlStatus/1  "ControlStatus"

== system Horizontal1804/IMUSensor/JapaneseExplanation ==

== system Horizontal1804/JoystickFeedback40/JapaneseExplanation ==

== system Horizontal1804/MagnetometerSensor/JapaneseExplanation ==

== system Horizontal1804/MotorWrite/JapaneseExplanation ==

== system Horizontal1804/OpticalFlowDistance50/JapaneseExplanation ==

== system Horizontal1804/OpticalFlowSensor/JapaneseExplanation ==

== system Horizontal1804/SensorCorrection/IMUAxisConversion ==
  AccelMps2 : Inport
  GyroRps : Inport  Port=2
  AccelBodySigns : Product  Description=AccelBodySigns：入力の乗算・除算（**）を行います。フィルターは既存の演算順序を保ちます。  Inputs=**
  AccelToG : Product  Description=AccelToG：入力の乗算・除算（*/）を行います。フィルターは既存の演算順序を保ちます。  Inputs=*/
  BodyAxisSigns : Constant  Description=BodyAxisSigns：固定値 single([1;1;-1]) を出力します。意味と単位は親の機能説明と信号名を参照します。  Value=single([1;1;-1])
  GravityMps2 : Constant  Description=GravityMps2：固定値 single(9.80665) を出力します。意味と単位は親の機能説明と信号名を参照します。  Value=single(9.80665)
  GyroBodySigns : Product  Description=GyroBodySigns：入力の乗算・除算（**）を行います。フィルターは既存の演算順序を保ちます。  Inputs=**
  JapaneseExplanation : Subsystem  Description=センサー XYZ を機体 [Y, X, -Z] へ変換します。加速度を m/s² から g 基準へ換算し、角速度は rad/s を保ちます。この座標変換はセンサーの取り付けと既存制御の定義に必要です。
      mask help: センサー XYZ を機体 [Y, X, -Z] へ変換します。加速度を m/s² から g 基準へ換算し、角速度は rad/s を保ちます。この座標変換はセンサーの取り付けと既存制御の定義に必要です。
      mask Display: disp(sprintf('センサー XYZ を機体 [Y, X, -Z] へ変換します。\n加速度を m/s² から g 基準へ換算し、角速度は rad/s を保ちます。\nこの座標変換はセンサーの取り付けと既存制御の定義に必要です。'));
  SwapAccelXY : Selector  Description=SwapAccelXY：必要なベクトル成分を選びます。選択位置は設定画面の Indices で確認します。  InputPortWidth=3  IndexOptions=Index vector (dialog)  Indices=[2 1 3]  OutputSizes=1
  SwapGyroXY : Selector  Description=SwapGyroXY：必要なベクトル成分を選びます。選択位置は設定画面の Indices で確認します。  InputPortWidth=3  IndexOptions=Index vector (dialog)  Indices=[2 1 3]  OutputSizes=1
  BodyAccelG : Outport
  BodyGyroRps : Outport  Port=2
  wires:
  BodyAxisSigns/1 -> AccelBodySigns/2, GyroBodySigns/2
  AccelMps2/1 -> SwapAccelXY/1
  AccelBodySigns/1 -> BodyAccelG/1
  AccelToG/1 -> AccelBodySigns/1
  GyroRps/1 -> SwapGyroXY/1
  GravityMps2/1 -> AccelToG/2
  SwapAccelXY/1 -> AccelToG/1
  SwapGyroXY/1 -> GyroBodySigns/1
  GyroBodySigns/1 -> BodyGyroRps/1

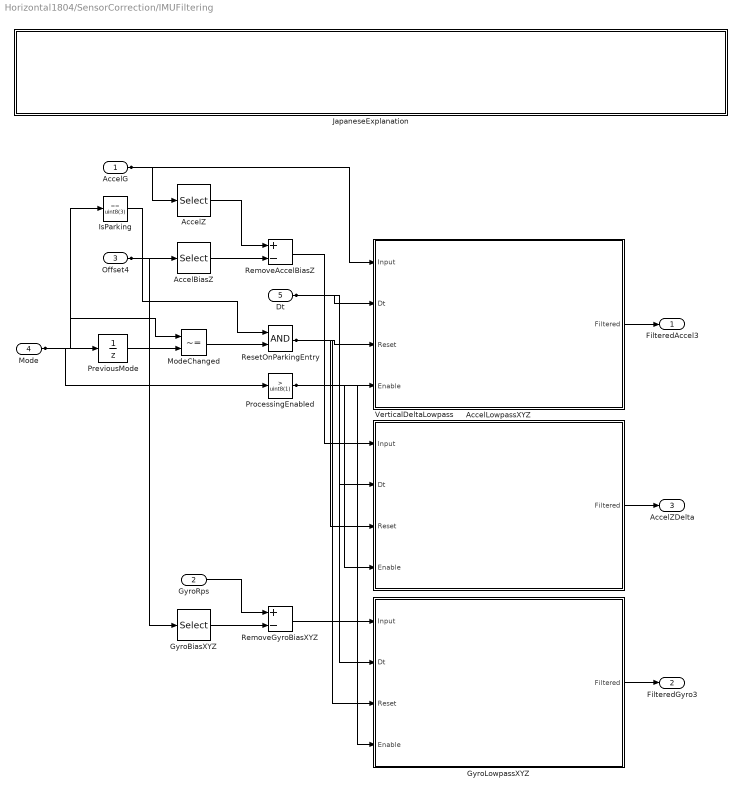
== system Horizontal1804/SensorCorrection/IMUFiltering ==
  AccelG : Inport
  GyroRps : Inport  Port=2
  Offset4 : Inport  Port=3
  Mode : Inport  Port=4
  Dt : Inport  Port=5
  AccelBiasZ : Selector  Description=AccelBiasZ：必要なベクトル成分を選びます。選択位置は設定画面の Indices で確認します。  InputPortWidth=4  IndexOptions=Index vector (dialog)  Indices=4  OutputSizes=1
  AccelLowpassXYZ : Subsystem  Description=加速度 XYZ の各成分へ同じ一次低域フィルターを適用します。状態と Reset の初期値は 3 要素です。式は s*T/(T+dt) + u*dt/(T+dt)。Enable=0 で保持します。
      mask help: 加速度 XYZ の各成分へ同じ一次低域フィルターを適用します。状態と Reset の初期値は 3 要素です。式は s*T/(T+dt) + u*dt/(T+dt)。Enable=0 で保持します。
      mask Display: disp('AccelLowpassXYZ');port_label('input',1,'Input');port_label('input',2,'Dt');port_label('input',3,'Reset');port_label('input',4,'Enable');port_label('output',1,'Filtered');
  AccelZ : Selector  Description=AccelZ：必要なベクトル成分を選びます。選択位置は設定画面の Indices で確認します。  InputPortWidth=3  IndexOptions=Index vector (dialog)  Indices=3  OutputSizes=1
  GyroBiasXYZ : Selector  Description=GyroBiasXYZ：必要なベクトル成分を選びます。選択位置は設定画面の Indices で確認します。  InputPortWidth=4  IndexOptions=Index vector (dialog)  Indices=[1 2 3]  OutputSizes=1
  GyroLowpassXYZ : Subsystem  Description=バイアス補正後の角速度 XYZ を成分ごとに平滑化します。順序と単位 rad/s を保ち、時定数 3 ms、実測 dt、Reset・Enable 条件を使います。
      mask help: バイアス補正後の角速度 XYZ を成分ごとに平滑化します。順序と単位 rad/s を保ち、時定数 3 ms、実測 dt、Reset・Enable 条件を使います。
      mask Display: disp('GyroLowpassXYZ');port_label('input',1,'Input');port_label('input',2,'Dt');port_label('input',3,'Reset');port_label('input',4,'Enable');port_label('output',1,'Filtered');
  IsParking : simulink/Logic and Bit Operations/Compare To Constant  relop===  const=uint8(3)  OutDataTypeStr=boolean
  JapaneseExplanation : Subsystem  Description=加速度と校正後角速度の XYZ ベクトルを時定数 3 ms で低域フィルターに通します。Z 加速度の校正差分は 100 ms で処理します。Mode 0, 1 の保持、待機への移行時リセット、実測 dt と既存の演算順序を維持します。
      mask help: 加速度と校正後角速度の XYZ ベクトルを時定数 3 ms で低域フィルターに通します。Z 加速度の校正差分は 100 ms で処理します。Mode 0, 1 の保持、待機への移行時リセット、実測 dt と既存の演算順序を維持します。
      mask Display: disp(sprintf('加速度と校正後角速度の XYZ ベクトルを時定数 3 ms で低域フィルターに通します。\nZ 加速度の校正差分は 100 ms で処理します。\nMode 0, 1 の保持、待機への移行時リセット、実測 dt と既存の演算順序を維持します。'));
  ModeChanged : RelationalOperator  Operator=~=  OutDataTypeStr=boolean  RndMeth=Simplest  InputSameDT=off
  PreviousMode : UnitDelay  Description=PreviousMode：前周期の値を保持して出力します。更新順序と状態保持に必要な 1 周期遅延です。初期値 uint8(0)、周期 .0025 秒。  InitialCondition=uint8(0)  SampleTime=.0025
  ProcessingEnabled : simulink/Logic and Bit Operations/Compare To Constant  relop=>  const=uint8(1)  OutDataTypeStr=boolean
  RemoveAccelBiasZ : Sum  Description=RemoveAccelBiasZ：入力を +- の符号で加減算します。ベクトルでは各成分に同じ演算を適用します。  Inputs=+-
  RemoveGyroBiasXYZ : Sum  Description=RemoveGyroBiasXYZ：入力を +- の符号で加減算します。ベクトルでは各成分に同じ演算を適用します。  Inputs=+-
  ResetOnParkingEntry : Logic  IconShape=distinctive  AllPortsSameDT=off  OutDataTypeStr=boolean
  VerticalDeltaLowpass : Subsystem  Description=校正後の加速度 Z 差分を時定数 100 ms で平滑化します。高度推定で使う従来の g 基準を保ちます。
      mask help: 校正後の加速度 Z 差分を時定数 100 ms で平滑化します。高度推定で使う従来の g 基準を保ちます。
      mask Display: disp('VerticalDeltaLowpass');port_label('input',1,'Input');port_label('input',2,'Dt');port_label('input',3,'Reset');port_label('input',4,'Enable');port_label('output',1,'Filtered');
  FilteredAccel3 : Outport
  FilteredGyro3 : Outport  Port=2
  AccelZDelta : Outport  Port=3
  wires:
  Mode/1 -> ModeChanged/1, PreviousMode/1, ProcessingEnabled/1, IsParking/1
  Offset4/1 -> AccelBiasZ/1, GyroBiasXYZ/1
  AccelG/1 -> AccelLowpassXYZ/1(Input), AccelZ/1
  PreviousMode/1 -> ModeChanged/2
  AccelZ/1 -> RemoveAccelBiasZ/1
  IsParking/1 -> ResetOnParkingEntry/1
  AccelBiasZ/1 -> RemoveAccelBiasZ/2
  ModeChanged/1 -> ResetOnParkingEntry/2
  GyroRps/1 -> RemoveGyroBiasXYZ/1
  ProcessingEnabled/1 -> VerticalDeltaLowpass/4(Enable), AccelLowpassXYZ/4(Enable), GyroLowpassXYZ/4(Enable)
  GyroBiasXYZ/1 -> RemoveGyroBiasXYZ/2
  RemoveAccelBiasZ/1 -> VerticalDeltaLowpass/1(Input)
  Dt/1 -> GyroLowpassXYZ/2(Dt), AccelLowpassXYZ/2(Dt), VerticalDeltaLowpass/2(Dt)
  ResetOnParkingEntry/1 -> VerticalDeltaLowpass/3(Reset), GyroLowpassXYZ/3(Reset), AccelLowpassXYZ/3(Reset)
  RemoveGyroBiasXYZ/1 -> GyroLowpassXYZ/1(Input)
  AccelLowpassXYZ/1(Filtered) -> FilteredAccel3/1
  VerticalDeltaLowpass/1(Filtered) -> AccelZDelta/1
  GyroLowpassXYZ/1(Filtered) -> FilteredGyro3/1

== system Horizontal1804/SensorCorrection/JapaneseExplanation ==

== system Horizontal1804/SensorCorrection/VerticalAcceleration ==
  AccelZDelta : Inport
  Mode : Inport  Port=2
  Dt : Inport  Port=3
  IsParking : simulink/Logic and Bit Operations/Compare To Constant  relop===  const=uint8(3)  OutDataTypeStr=boolean
  JapaneseExplanation : Subsystem  Description=校正後の Z 加速度差分の符号を反転し、上向きの鉛直加速度を作ります。100 ms の平滑化とモードによる保持・リセットを行います。高度 Kalman は従来の g 基準の数値を受けます。
      mask help: 校正後の Z 加速度差分の符号を反転し、上向きの鉛直加速度を作ります。100 ms の平滑化とモードによる保持・リセットを行います。高度 Kalman は従来の g 基準の数値を受けます。
      mask Display: disp(sprintf('校正後の Z 加速度差分の符号を反転し、上向きの鉛直加速度を作ります。\n100 ms の平滑化とモードによる保持・リセットを行います。\n高度 Kalman は従来の g 基準の数値を受けます。'));
  ModeChanged : RelationalOperator  Operator=~=  OutDataTypeStr=boolean  RndMeth=Simplest  InputSameDT=off
  PreviousMode : UnitDelay  Description=PreviousMode：前周期の値を保持して出力します。更新順序と状態保持に必要な 1 周期遅延です。初期値 uint8(0)、周期 .0025 秒。  InitialCondition=uint8(0)  SampleTime=.0025
  ProcessingEnabled : simulink/Logic and Bit Operations/Compare To Constant  relop=>  const=uint8(1)  OutDataTypeStr=boolean
  ResetOnParkingEntry : Logic  IconShape=distinctive  AllPortsSameDT=off  OutDataTypeStr=boolean
  UpwardSign : Gain  Description=UpwardSign：入力に single(-1) を掛けます。座標変換・単位換算・制御係数は用途ごとに維持します。  Gain=single(-1)
  VerticalLowpass : Subsystem  Description=鉛直加速度の一次低域フィルターです。実測 dt、時定数 100 ms、Enable と Reset の条件を使って前回値を更新します。
      mask help: 鉛直加速度の一次低域フィルターです。実測 dt、時定数 100 ms、Enable と Reset の条件を使って前回値を更新します。
      mask Display: disp('VerticalLowpass');port_label('input',1,'Input');port_label('input',2,'Dt');port_label('input',3,'Reset');port_label('input',4,'Enable');port_label('output',1,'Filtered');
  VerticalAccel : Outport
  wires:
  ProcessingEnabled/1 -> VerticalLowpass/4(Enable)
  Mode/1 -> ProcessingEnabled/1, PreviousMode/1, ModeChanged/1, IsParking/1
  PreviousMode/1 -> ModeChanged/2
  IsParking/1 -> ResetOnParkingEntry/1
  Dt/1 -> VerticalLowpass/2(Dt)
  ModeChanged/1 -> ResetOnParkingEntry/2
  AccelZDelta/1 -> UpwardSign/1
  UpwardSign/1 -> VerticalLowpass/1(Input)
  ResetOnParkingEntry/1 -> VerticalLowpass/3(Reset)
  VerticalLowpass/1(Filtered) -> VerticalAccel/1

== system Horizontal1804/AttitudeAltitudeEstimation/IMUAttitude/FusionState ==
  Accel : Inport  PortDimensions=[1 3]
  Gyro : Inport  Port=2  PortDimensions=[1 3]
  Reset : Inport  Port=3
  Enable : EnablePort
  UpdateWhenReady : Subsystem  Description=標準 IMU Filter の状態へ再開時のリセットを適用する Resettable subsystem です。外側の Enabled 境界と役割が異なるため、この階層を保ちます。
      mask help: 標準 IMU Filter の状態へ再開時のリセットを適用する Resettable subsystem です。外側の Enabled 境界と役割が異なるため、この階層を保ちます。
      mask Display: disp('UpdateWhenReady');port_label('input',1,'Accel');port_label('input',2,'Gyro');port_label('output',1,'Orientation');port_label('output',2,'AngularVelocity');
  Orientation : Outport  PortDimensions=[1 4]  InitialOutput=single([1 0 0 0])
  AngularVelocity : Outport  Port=2  PortDimensions=[1 3]  InitialOutput=single([0 0 0])
  wires:
  UpdateWhenReady/2(AngularVelocity) -> AngularVelocity/1
  UpdateWhenReady/1(Orientation) -> Orientation/1
  Gyro/1 -> UpdateWhenReady/2(Gyro)
  Accel/1 -> UpdateWhenReady/1(Accel)
  Reset/1 -> UpdateWhenReady/Reset

== system Horizontal1804/FlightControl/TakeoffHoverControl/AltitudeControl ==
  VerticalEstimate : Inport
  AltitudeCommand : Inport  Port=2
  AltitudeContext : Inport  Port=3
  AltitudeCommandFields : BusSelector  Description=AltitudeCommandFields：バスから HeightReference,BaseThrust,AltitudeEnabled,ManualAltitude を選びます。元のベクトルの成分順序は変更しません。  OutputSignals=HeightReference,BaseThrust,AltitudeEnabled,ManualAltitude
  AltitudeContextFields : BusSelector  Description=制御の実行・リセット条件と実測 dt を選びます。DedicatedPID 内部で前回誤差を保持するため、未使用の PreviousError は取り出しません。  OutputSignals=ThrustRequest,ControlContext.VelocityEnabled,ControlContext.AltitudeEnabled,ControlContext.Reset,FlightContext.Branch,Mode,Dt
  AltitudeError : Sum  Description=AltitudeError：入力を +- の符号で加減算します。ベクトルでは各成分に同じ演算を適用します。  Inputs=+-
  AltitudePID : Subsystem  Description=高度 PID：高度誤差→鉛直速度目標。Enabled subsystem が状態更新を許可し、低推力 Reset が積分・微分状態を初期化します。内部 DedicatedPID は Ideal・離散・台形積分/微分・外部 dt です。P=0.38、I=0.1、D=0.5、N=16。
      mask help: 高度 PID：高度誤差→鉛直速度目標。Enabled subsystem が状態更新を許可し、低推力 Reset が積分・微分状態を初期化します。内部 DedicatedPID は Ideal・離散・台形積分/微分・外部 dt です。P=0.38、I=0.1、D=0.5、N=16。
      mask Display: disp('AltitudePID');port_label('input',1,'Error');port_label('input',2,'Dt');port_label('input',3,'Reset');port_label('output',1,'Output');
  HeldThrustMemory : UnitDelay  Description=HeldThrustMemory：前周期の値を保持して出力します。更新順序と状態保持に必要な 1 周期遅延です。初期値 single(0)、周期 Official.Step 秒。  InitialCondition=single(0)  SampleTime=Official.Step
  SelectVerticalReference : MATLAB Function  Description=鉛直速度目標を選びます。Auto Altitude 時は高度 PID の目標を使い、手動高度で着陸中（Mode 5）のときだけ -0.15 の降下目標に切り替えます。  TreatAsAtomicUnit=on
  ThrustCorrectionLimits : MATLAB Function  Description=共通推力を決めます。鉛直速度 PID の補正を基準推力へ加え、10 ms で平滑化します。Auto Altitude 時は基準の 0.85～1.15 倍に制限し、指定された分岐では前回推力を保持します。  TreatAsAtomicUnit=on
  ThrustFilterMemory : UnitDelay  Description=ThrustFilterMemory：前周期の値を保持して出力します。更新順序と状態保持に必要な 1 周期遅延です。初期値 single(0)、周期 Official.Step 秒。  InitialCondition=single(0)  SampleTime=Official.Step
  ThrustStateBus : BusCreator  Description=ThrustStateBus：異なる単位・型を持つ関連信号を名前付きバスにまとめます。入力線の信号名が項目名です。  Inputs=2
  VerticalEstimateFields : BusSelector  Description=VerticalEstimateFields：バスから Altitude,Velocity を選びます。元のベクトルの成分順序は変更しません。  OutputSignals=Altitude,Velocity
  VerticalSpeedError : Sum  Description=VerticalSpeedError：入力を +- の符号で加減算します。ベクトルでは各成分に同じ演算を適用します。  Inputs=+-
  VerticalSpeedPID : Subsystem  Description=鉛直速度 PID：速度誤差→基準推力の補正。Enabled 境界・外部 Reset・実測 dt と既存係数を保持します。内部の DedicatedPID で係数を設定します。
      mask help: 鉛直速度 PID：速度誤差→基準推力の補正。Enabled 境界・外部 Reset・実測 dt と既存係数を保持します。内部の DedicatedPID で係数を設定します。
      mask Display: disp('VerticalSpeedPID');port_label('input',1,'Error');port_label('input',2,'Dt');port_label('input',3,'Reset');port_label('output',1,'Output');
  Thrust : Outport
  VerticalReference : Outport  Port=2
  ThrustState : Outport  Port=3
  wires:
  AltitudeContext/1 -> AltitudeContextFields/1
  AltitudeCommandFields/4 -> ThrustCorrectionLimits/5(arg_arg_manual)  "<ManualAltitude>"
  AltitudeCommandFields/2 -> ThrustCorrectionLimits/3(arg_arg_base)  "<BaseThrust>"
  VerticalEstimate/1 -> VerticalEstimateFields/1
  AltitudeCommand/1 -> AltitudeCommandFields/1
  AltitudeCommandFields/3 -> SelectVerticalReference/3(arg_auto), ThrustCorrectionLimits/4(arg_arg_auto)  "<AltitudeEnabled>"
  AltitudeCommandFields/1 -> AltitudeError/1  "<HeightReference>"
  VerticalEstimateFields/1 -> AltitudeError/2  "<Altitude>"
  VerticalEstimateFields/2 -> VerticalSpeedError/2  "<Velocity>"
  AltitudeError/1 -> AltitudePID/1(Error)
  AltitudePID/1(Output) -> SelectVerticalReference/1(arg_zRef), VerticalReference/1  "VelocityReference"
  AltitudeContextFields/1 -> ThrustCorrectionLimits/1(arg_arg_command)  "<ThrustRequest>"
  SelectVerticalReference/1(arg_vRef) -> VerticalSpeedError/1
  AltitudeContextFields/2 -> VerticalSpeedPID/Enable, ThrustCorrectionLimits/6(arg_arg_velEnable)  "<VelocityEnabled>"
  AltitudeContextFields/3 -> AltitudePID/Enable  "<AltitudeEnabled>"
  AltitudeContextFields/4 -> AltitudePID/3(Reset), VerticalSpeedPID/3(Reset)  "<Reset>"
  AltitudeContextFields/5 -> ThrustCorrectionLimits/7(arg_branch)  "<Branch>"
  AltitudeContextFields/6 -> SelectVerticalReference/2(arg_mode)  "<Mode>"
  AltitudeContextFields/7 -> ThrustCorrectionLimits/8(arg_arg_dt), VerticalSpeedPID/2(Dt), AltitudePID/2(Dt)  "<Dt>"
  VerticalSpeedError/1 -> VerticalSpeedPID/1(Error)
  VerticalSpeedPID/1(Output) -> ThrustCorrectionLimits/2(arg_arg_correction)
  ThrustFilterMemory/1 -> ThrustStateBus/1, ThrustCorrectionLimits/9(arg_arg_oldFilter)  "FilteredThrust"
  ThrustCorrectionLimits/1(arg_arg_thrust) -> Thrust/1  "Thrust"
  ThrustCorrectionLimits/2(arg_arg_filter) -> ThrustFilterMemory/1
  ThrustCorrectionLimits/3(arg_arg_last) -> HeldThrustMemory/1
  HeldThrustMemory/1 -> ThrustCorrectionLimits/10(arg_arg_lastThrust), ThrustStateBus/2  "HeldThrust"
  ThrustStateBus/1 -> ThrustState/1  "ThrustState"
